simulink subsystem "controller"  (R2026a)
settings: Solver=VariableStepAuto
undefined symbols (not defined in the file): S
PreSaveFcn:
  | defaultToFileBlockNames(bdroot);
settings Model: Creator=koryh  LastModifiedBy=kjhaydon

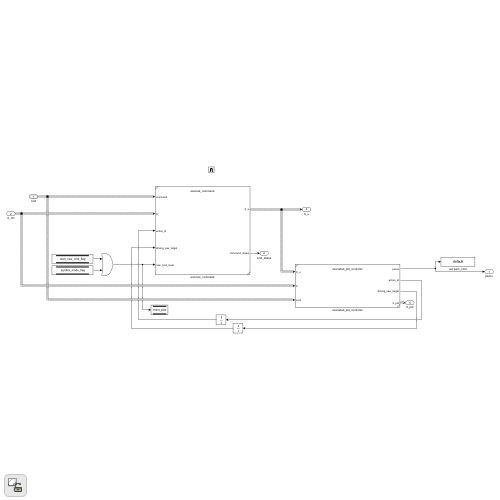
[thumbnail: Simulink's stored preview of the top-level diagram]
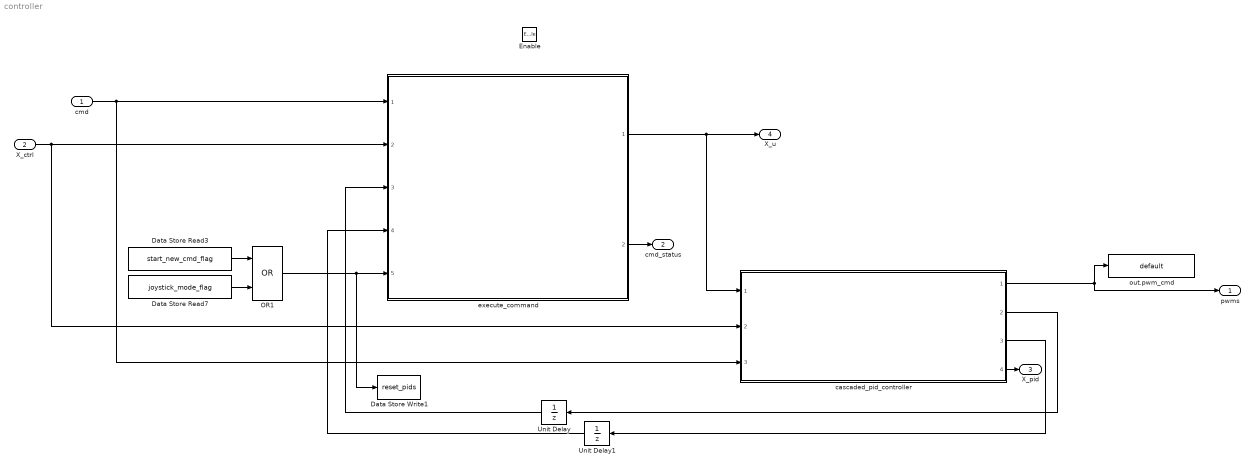
== system controller ==
  cmd : Inport  OutDataTypeStr=Bus: cmd_bus  SampleTime=S.dt_control
      settings: VarSizeSig=Yes
  X_ctrl : Inport  Port=2  SampleTime=S.dt_control
  Enable : EnablePort
  Data Store Read3 : DataStoreRead  DataStoreName=start_new_cmd_flag  IndexOptions=Index vector (dialog)  Indices=1  OutputSizes=1
  Data Store Read7 : DataStoreRead  DataStoreName=joystick_mode_flag  IndexOptions=Index vector (dialog)  Indices=1  OutputSizes=1
  Data Store Write1 : DataStoreWrite  DataStoreName=reset_pids  IndexOptions=Index vector (dialog)  Indices=1  OutputSizes=1
  OR1 : Logic  Operator=OR  IconShape=distinctive  AllPortsSameDT=off  OutDataTypeStr=boolean
  Unit Delay : UnitDelay  SampleTime=S.dt_control
  Unit Delay1 : UnitDelay  SampleTime=S.dt_control
  cascaded_pid_controller : Subsystem  ReferencedSubsystem=cascaded_pid_controller
  execute_command : Subsystem  ReferencedSubsystem=execute_command
  out.pwm_cmd : ToFile  Filename=default  MatrixName=pwm_cmd  SaveFormat=Timeseries  SampleTime=S.dt_data
  pwms : Outport
  cmd_status : Outport  Port=2  SampleTime=S.dt_control
  X_pid : Outport  Port=3
  X_u : Outport  Port=4
  wires:
  X_ctrl/1 -> cascaded_pid_controller/2, execute_command/2
  cascaded_pid_controller/1 -> out.pwm_cmd/1, pwms/1
  cascaded_pid_controller/2 -> Unit Delay/1
  Unit Delay/1 -> execute_command/3
  cascaded_pid_controller/3 -> Unit Delay1/1
  execute_command/2 -> cmd_status/1
  cmd/1 -> cascaded_pid_controller/3, execute_command/1
  Unit Delay1/1 -> execute_command/4
  Data Store Read3/1 -> OR1/1
  execute_command/1 -> cascaded_pid_controller/1, X_u/1
  Data Store Read7/1 -> OR1/2
  OR1/1 -> execute_command/5, Data Store Write1/1
  cascaded_pid_controller/4 -> X_pid/1
